simulink model "pioneerSNL"  (R2023b)
settings: Solver=ode23t  StartTime=0  StopTime=1300  FixedStep=0.05  MaxStep=0.05  RelTol=1e-3
values from neighbouring files (symbols this model uses):
  aboveWaterMass = 0    [wecSimInputFile.m]
  L0 = 15+19.8    (= 34.8)    [buildMCR.m]    (also in wecSimInputFile.m)
  polyNom = 1.0e+04*[1.9488   -0.0390   -1.3588    0.8094   -0.0004]    [wecSimInputFile.m]
  simu = simulationClass()    [wecSimInputFile.m]
  waves = waveClass('spectrumImportFullDir')    [wecSimInputFile.m]
undefined symbols (not defined in the file or in its folder): body, cable, constraint, geometry, hydroData, pto, X, Y, Z
libraries: nesl_utility x21, sm_lib x17, WECSim_Lib_Body_Elements x7, WECSim_Lib_PTOs x3, WECSim_Lib_Constraints x2, WECSim_Lib_Cables x1, WECSim_Lib_Moorings x1, WECSim_Lib_Frames x1
(part 1 of 2)
settings Model: Creator=dforbus  LastModifiedBy=jtgrasb
settings SolverCC: ZeroCrossControl=DisableAll  AutoInsertRateTranBlk=on
settings DataIOCC: ReturnWorkspaceOutputs=off
settings OptimizationCC: SimCompilerOptimization=on

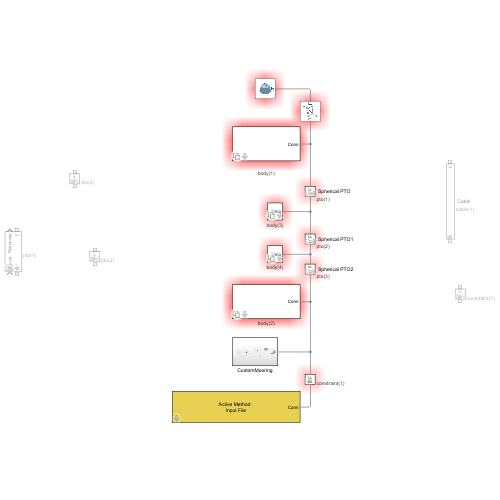
[thumbnail: Simulink's stored preview of the top-level diagram]
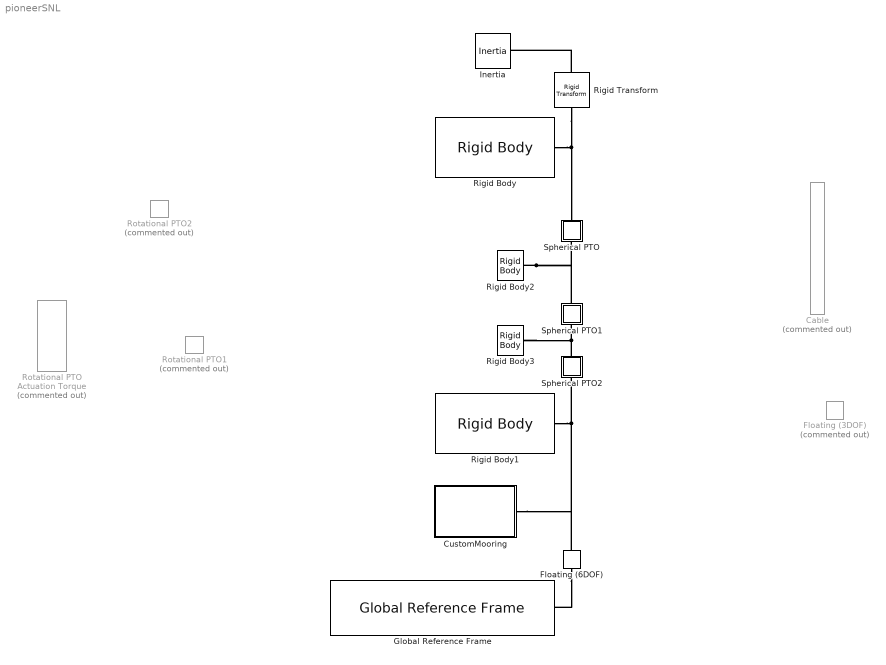
== system pioneerSNL ==
  Cable : WECSim_Lib_Cables/Cable  Commented=on  VariantControl=sv_Cable3DOF  cable=cable(1)  baseConnectionName=constraint(1)  followerConnectionName=constraint(2)  stiffness=0  damping=0  length=0  preTension=0  diplacement=0 0 0  axis=0 1 0  angle=0  y=0 1 0  z=0 0 1
      settings: AttributesFormatString=%<cable>
  CustomMooring : Subsystem
  Floating (3DOF) : WECSim_Lib_Constraints/Floating (3DOF)  Commented=on  constraint=constraint(1)  loc="0  0  0"  displacement=0 0 0  y=0 1 0  z=0 0 1  upperLimitSpecify=off  upperLimitBound=0  upperLimitTransitionRegionWidth=0  upperLimitStiffness=0  upperLimitDamping=0  lowerLimitSpecify=off  lowerLimitBound=0  lowerLimitTransitionRegionWidth=0  lowerLimitStiffness=0  lowerLimitDamping=0
      settings: AttributesFormatString=%<constraint>
  Floating (6DOF) : WECSim_Lib_Constraints/Floating (6DOF)  constraint=constraint(1)  loc="0  0  0"  displacement=0 0 0  y=0 1 0  z=0 0 1  upperLimitSpecify=off  upperLimitBound=0  upperLimitTransitionRegionWidth=0  upperLimitStiffness=0  upperLimitDamping=0  lowerLimitSpecify=off  lowerLimitBound=0  lowerLimitTransitionRegionWidth=0  lowerLimitStiffness=0  lowerLimitDamping=0
      settings: AttributesFormatString=%<constraint>
  Global Reference Frame : WECSim_Lib_Frames/Global Reference Frame  waves=waves  simu=simu  InputMethod=Input File  InputFile=wecSimInputFile.m  mode=normal  explorer=off  solver=ode4  startTime=0  rampTime=100  endTime=400  dt=0.1  cicEndTime=60  stateSpace=0  WaveClass=regular  height=2.5  period=8  elevationFile=NOT DEFINED  spectrumFile=NOT DEFINED  direction=0  spread=1  spectrumType=NOT DEFINED  phaseSeed=0  option=EqualEnergy
  Inertia : sm_lib/Body Elements/Inertia  InertiaType=PointMass  Mass=aboveWaterMass  MassUnits=kg  CenterOfMass=[0 0 0]  CenterOfMassUnits=m  MomentsOfInertia=[1 1 1]  MomentsOfInertiaUnits=kg*m^2  ProductsOfInertia=[0 0 0]  ProductsOfInertiaUnits=kg*m^2  GraphicType=Marker  MarkerShape=Inertia  MarkerSize=20  GraphicVisPropType=SimpleVisualProperties  GraphicDiffuseColor=[0.5 0.5 0.5]  GraphicSpecularColor=[0.5 0.5 0.5 1.0]  GraphicAmbientColor=[0.15 0.15 0.15 1.0]  GraphicEmissiveColor=[0.0 0.0 0.0 1.0]  GraphicShininess=75  GraphicOpacity=1.0
  Rigid Transform : sm_lib/Frames and Transforms/Rigid Transform  TranslationMethod=Cartesian  TranslationStandardOffset=0  TranslationStandardOffsetUnits=m  TranslationStandardAxis=+Z  TranslationCartesianOffset=aboveWaterMassLoc  TranslationCartesianOffsetUnits=m  TranslationROffset=0  TranslationROffsetUnits=m  TranslationZOffset=0  TranslationZOffsetUnits=m  TranslationThetaOffset=0  TranslationThetaOffsetUnits=deg  RotationMethod=None  RotationAngleUnits=deg  RotationStandardAxis=+Z  RotationAngle=0.0  RotationArbitraryAxis=[0 0 1]  FollAlignAxisA=+X  BaseAlignAxisA=+Y  FollAlignAxisB=+Y  BaseAlignAxisB=+Z  RotationSequenceAxes=FollowerAxes  RotationSequence=XYX  RotationSequenceAngles=[0 0 0]  RotationSequenceAnglesUnits=deg  RotationMatrix=[1 0 0; 0 1 0; 0 0 1]  Quaternion=[1 0 0 0]
  Rigid Body : WECSim_Lib_Body_Elements/Rigid Body  body=body(1)  h5File=hydroData/*.h5  geometryFile=geometry/*.stl  mass=0  inertia=0 0 0  inertiaProducts=0 0 0  nonHydro=0  nonlinearHydro=0  centerGravity=0 0 0  centerBuoyancy=0 0 0  dof=6  volume=0  QTFs=0  displacement=0 0 0  axis=0 1 0  angle=0  option=0  cd=0 0 0  ca=0 0 0  area=0 0 0  VME=0  rgME=0 0 0  z=0 0 1
  Rigid Body1 : WECSim_Lib_Body_Elements/Rigid Body  body=body(2)  h5File=hydroData/*.h5  geometryFile=geometry/*.stl  mass=0  inertia=0 0 0  inertiaProducts=0 0 0  nonHydro=0  nonlinearHydro=0  centerGravity=0 0 0  centerBuoyancy=0 0 0  dof=6  volume=0  QTFs=0  displacement=0 0 0  axis=0 1 0  angle=0  option=0  cd=0 0 0  ca=0 0 0  area=0 0 0  VME=0  rgME=0 0 0  z=0 0 1
  Rigid Body2 : WECSim_Lib_Body_Elements/Rigid Body  body=body(3)  h5File=hydroData/*.h5  geometryFile=geometry/*.stl  mass=0  inertia=0 0 0  inertiaProducts=0 0 0  nonHydro=0  nonlinearHydro=0  centerGravity=0 0 0  centerBuoyancy=0 0 0  dof=6  volume=0  QTFs=0  displacement=0 0 0  axis=0 1 0  angle=0  option=0  cd=0 0 0  ca=0 0 0  area=0 0 0  VME=0  rgME=0 0 0  z=0 0 1
  Rigid Body3 : WECSim_Lib_Body_Elements/Rigid Body  body=body(4)  h5File=hydroData/*.h5  geometryFile=geometry/*.stl  mass=0  inertia=0 0 0  inertiaProducts=0 0 0  nonHydro=0  nonlinearHydro=0  centerGravity=0 0 0  centerBuoyancy=0 0 0  dof=6  volume=0  QTFs=0  displacement=0 0 0  axis=0 1 0  angle=0  option=0  cd=0 0 0  ca=0 0 0  area=0 0 0  VME=0  rgME=0 0 0  z=0 0 1
  Rotational PTO Actuation Torque : WECSim_Lib_PTOs/Rotational PTO Actuation Torque  Commented=on  pto=pto(1)  loc="0  0  0"  stiffness=0  damping=0  equilibriumPosition=0  pretension=0  displacement=0 0 0  y=0 1 0  z=0 0 1  upperLimitSpecify=off  upperLimitBound=0  upperLimitTransitionRegionWidth=0  upperLimitStiffness=0  upperLimitDamping=0  lowerLimitSpecify=off  lowerLimitBound=0  lowerLimitTransitionRegionWidth=0  lowerLimitStiffness=0  lowerLimitDamping=0
      settings: AttributesFormatString=%<pto>
  Rotational PTO1 : WECSim_Lib_PTOs/Rotational PTO  Commented=on  pto=pto(2)  loc="0  0  0"  stiffness=0  damping=0  equilibriumPosition=0  pretension=0  displacement=0 0 0  y=0 1 0  z=0 0 1  upperLimitSpecify=off  upperLimitBound=0  upperLimitTransitionRegionWidth=0  upperLimitStiffness=0  upperLimitDamping=0  lowerLimitSpecify=off  lowerLimitBound=0  lowerLimitTransitionRegionWidth=0  lowerLimitStiffness=0  lowerLimitDamping=0
      settings: AttributesFormatString=%<pto>
  Rotational PTO2 : WECSim_Lib_PTOs/Rotational PTO  Commented=on  pto=pto(3)  loc="0  0  0"  stiffness=0  damping=0  equilibriumPosition=0  pretension=0  displacement=0 0 0  y=0 1 0  z=0 0 1  upperLimitSpecify=off  upperLimitBound=0  upperLimitTransitionRegionWidth=0  upperLimitStiffness=0  upperLimitDamping=0  lowerLimitSpecify=off  lowerLimitBound=0  lowerLimitTransitionRegionWidth=0  lowerLimitStiffness=0  lowerLimitDamping=0
      settings: AttributesFormatString=%<pto>
  Spherical PTO : Subsystem  AncestorBlock=WECSim_Lib_PTOs/Spherical PTO  mask(PTOs){pto=pto(1), InputFileText=Global Reference Frame option "Use Input File" is selected., loc=[0 0 0], stiffness=0, damping=0, displacement=[0 0 0], x=, y=0 1 0, z=0 0 1, upperLimitSpecify=on, upperLimitBound=0, upperLimitTransitionRegionWidth=0, upperLimitStiffness=0, upperLimitDamping=0, lowerLimitSpecify=on, lowerLimitBound=0, lowerLimitTransitionRegionWidth=0, lowerLimitStiffness=0, lowerLimitDamping=0}
      mask prompts: pto "PTO Name:"; loc "Location [m]:"; stiffness "PTO Stiffness [N/m]"; damping "PTO Damping [N/m/s]"; displacement "Initial linear displacement [m]:"; x "X-axis [m]:"; y "Y-axis [m]:"; z "Z-axis [m]:"; upperLimitSpecify "Upper limit"; upperLimitBound "Upper limit bound [m, deg]"; upperLimitTransitionRegionWidth "Upper limit transition region width [m, deg]:"; upperLimitStiffness "Upper limit stiffness [N/m, Nm/rad]:"; upperLimitDamping "Upper limit damping [N/(m/s), Nm/(rad/s)]:"; lowerLimitSpecify "Lower limit"; lowerLimitBound "Lower limit bound [m, deg]:"; lowerLimitTransitionRegionWidth "Lower limit transition region width [m, deg]:"; lowerLimitStiffness "Lower limit stiffness [N/m, Nm/rad]:"; lowerLimitDamping "Lower limit damping [N/(m/s), Nm/(rad/s)]:"
      mask help:
      | Constrains the follower to rotational motion relative to the base, fixing in
      | X,Y,Z but allowing rotation about each axis and adds PTO stiffness and damping.
      |
      | The variable name input below must be 'pto(i)' where i=1,2,...
      | pto(i) must be defined in the input file with the following fields:
      |
      |     .name (required)
      |             String.
      |            Constraint name. Must comply with Matlab's variable naming rules.
      |     .location (optional)
      |             3x1 vector [x y z] in meters.
      |             Constraint location. Default = [0 0 0]
      |     .stiffness (optional)
      |             Float.
      |             PTO linear spring stiffness. Default = 0
      |     .damping (optional)
      |             Float.
      |             PTO linear damping coefficient. Default = 0
      |     .orientation.z (optional)
      |             3x1 vector [x y z].
      |             Direction of the constraint's Z-coordinate. Default = [0 0 1]
      |     .orientation.y (optional)
      |             3x1 vector [x y z].
      |             Direction of the constraint's Y-coordinate. Default = [0 1 0]
      mask init:
      | if exist('pto','var')
      |     h=[gcb '/To Workspace'];
      |     responseName=['pto' num2str(pto.number) '_out'];
      |     set_param(h,'VariableName',responseName);
      |     h=[gcb '/Spherical Joint)'];
      |     try % this should catch any version issue for which these parameters do not exist
      |         set_param(h,'upperLimitSpecify',pto.hardStops.upperLimitSpecify)
      |         set_param(h,'lowerLimitSpecify',pto.hardStops.lowerLimitSpecify)
      |     end
      | end
      | 
      | pto.checkLoc('W');
      settings: AttributesFormatString=%<pto>
      mask Help:
      | Constrains the follower to rotational motion relative to the base, fixing in
      | X,Y,Z but allowing rotation about each axis and adds PTO stiffness and damping.
      | 
      | The variable name input below must be 'pto(i)' where i=1,2,...
      | pto(i) must be defined in the input file with the following fields:
      | 
      |     .name (required)
      |             String.
      |            Constraint name. Must comply with Matlab's variable naming rules.
      |     .location (optional)
      |             3x1 vector [x y z] in meters.
      |             Constraint location. Default = [0 0 0]
      |     .stiffness (optional)
      |             Float.
      |             PTO linear spring stiffness. Default = 0
      |     .damping (optional)
      |             Float.
      |             PTO linear damping coefficient. Default = 0
      |     .orientation.z (optional)
      |             3x1 vector [x y z].
      |             Direction of the constraint's Z-coordinate. Default = [0 0 1]
      |     .orientation.y (optional)
      |             3x1 vector [x y z].
      |             Direction of the constraint's Y-coordinate. Default = [0 1 0]
      mask Callback upperLimitSpecify: hardStopCallback(gcbh)
      mask Callback lowerLimitSpecify: hardStopCallback(gcbh)
      mask DialogControl InputFileGroup Prompt: Input File
      mask DialogControl CustomParameterGroup Prompt: Custom Parameters
      mask DialogControl std_opts Prompt: Standard options
      mask DialogControl orientations Prompt: Orientation
      mask DialogControl Container7 Prompt: Hard stop
  Spherical PTO1 : Subsystem  AncestorBlock=WECSim_Lib_PTOs/Spherical PTO  mask(PTOs){pto=pto(2), InputFileText=Global Reference Frame option "Use Input File" is selected., loc=[0 0 0], stiffness=0, damping=0, displacement=[0 0 0], x=, y=0 1 0, z=0 0 1, upperLimitSpecify=on, upperLimitBound=0, upperLimitTransitionRegionWidth=0, upperLimitStiffness=0, upperLimitDamping=0, lowerLimitSpecify=on, lowerLimitBound=0, lowerLimitTransitionRegionWidth=0, lowerLimitStiffness=0, lowerLimitDamping=0}
      mask prompts: pto "PTO Name:"; loc "Location [m]:"; stiffness "PTO Stiffness [N/m]"; damping "PTO Damping [N/m/s]"; displacement "Initial linear displacement [m]:"; x "X-axis [m]:"; y "Y-axis [m]:"; z "Z-axis [m]:"; upperLimitSpecify "Upper limit"; upperLimitBound "Upper limit bound [m, deg]"; upperLimitTransitionRegionWidth "Upper limit transition region width [m, deg]:"; upperLimitStiffness "Upper limit stiffness [N/m, Nm/rad]:"; upperLimitDamping "Upper limit damping [N/(m/s), Nm/(rad/s)]:"; lowerLimitSpecify "Lower limit"; lowerLimitBound "Lower limit bound [m, deg]:"; lowerLimitTransitionRegionWidth "Lower limit transition region width [m, deg]:"; lowerLimitStiffness "Lower limit stiffness [N/m, Nm/rad]:"; lowerLimitDamping "Lower limit damping [N/(m/s), Nm/(rad/s)]:"
      mask help:
      | Constrains the follower to rotational motion relative to the base, fixing in
      | X,Y,Z but allowing rotation about each axis and adds PTO stiffness and damping.
      |
      | The variable name input below must be 'pto(i)' where i=1,2,...
      | pto(i) must be defined in the input file with the following fields:
      |
      |     .name (required)
      |             String.
      |            Constraint name. Must comply with Matlab's variable naming rules.
      |     .location (optional)
      |             3x1 vector [x y z] in meters.
      |             Constraint location. Default = [0 0 0]
      |     .stiffness (optional)
      |             Float.
      |             PTO linear spring stiffness. Default = 0
      |     .damping (optional)
      |             Float.
      |             PTO linear damping coefficient. Default = 0
      |     .orientation.z (optional)
      |             3x1 vector [x y z].
      |             Direction of the constraint's Z-coordinate. Default = [0 0 1]
      |     .orientation.y (optional)
      |             3x1 vector [x y z].
      |             Direction of the constraint's Y-coordinate. Default = [0 1 0]
      mask init: same as pioneerSNL/Spherical PTO
      settings: AttributesFormatString=%<pto>
      mask Help:
      | Constrains the follower to rotational motion relative to the base, fixing in
      | X,Y,Z but allowing rotation about each axis and adds PTO stiffness and damping.
      | 
      | The variable name input below must be 'pto(i)' where i=1,2,...
      | pto(i) must be defined in the input file with the following fields:
      | 
      |     .name (required)
      |             String.
      |            Constraint name. Must comply with Matlab's variable naming rules.
      |     .location (optional)
      |             3x1 vector [x y z] in meters.
      |             Constraint location. Default = [0 0 0]
      |     .stiffness (optional)
      |             Float.
      |             PTO linear spring stiffness. Default = 0
      |     .damping (optional)
      |             Float.
      |             PTO linear damping coefficient. Default = 0
      |     .orientation.z (optional)
      |             3x1 vector [x y z].
      |             Direction of the constraint's Z-coordinate. Default = [0 0 1]
      |     .orientation.y (optional)
      |             3x1 vector [x y z].
      |             Direction of the constraint's Y-coordinate. Default = [0 1 0]
      mask Callback upperLimitSpecify: hardStopCallback(gcbh)
      mask Callback lowerLimitSpecify: hardStopCallback(gcbh)
      mask DialogControl InputFileGroup Prompt: Input File
      mask DialogControl CustomParameterGroup Prompt: Custom Parameters
      mask DialogControl std_opts Prompt: Standard options
      mask DialogControl orientations Prompt: Orientation
      mask DialogControl Container7 Prompt: Hard stop
  Spherical PTO2 : Subsystem  AncestorBlock=WECSim_Lib_PTOs/Spherical PTO  mask(PTOs){pto=pto(3), InputFileText=Global Reference Frame option "Use Input File" is selected., loc=[0 0 0], stiffness=0, damping=0, displacement=[0 0 0], x=, y=0 1 0, z=0 0 1, upperLimitSpecify=on, upperLimitBound=0, upperLimitTransitionRegionWidth=0, upperLimitStiffness=0, upperLimitDamping=0, lowerLimitSpecify=on, lowerLimitBound=0, lowerLimitTransitionRegionWidth=0, lowerLimitStiffness=0, lowerLimitDamping=0}
      mask prompts: pto "PTO Name:"; loc "Location [m]:"; stiffness "PTO Stiffness [N/m]"; damping "PTO Damping [N/m/s]"; displacement "Initial linear displacement [m]:"; x "X-axis [m]:"; y "Y-axis [m]:"; z "Z-axis [m]:"; upperLimitSpecify "Upper limit"; upperLimitBound "Upper limit bound [m, deg]"; upperLimitTransitionRegionWidth "Upper limit transition region width [m, deg]:"; upperLimitStiffness "Upper limit stiffness [N/m, Nm/rad]:"; upperLimitDamping "Upper limit damping [N/(m/s), Nm/(rad/s)]:"; lowerLimitSpecify "Lower limit"; lowerLimitBound "Lower limit bound [m, deg]:"; lowerLimitTransitionRegionWidth "Lower limit transition region width [m, deg]:"; lowerLimitStiffness "Lower limit stiffness [N/m, Nm/rad]:"; lowerLimitDamping "Lower limit damping [N/(m/s), Nm/(rad/s)]:"
      mask help:
      | Constrains the follower to rotational motion relative to the base, fixing in
      | X,Y,Z but allowing rotation about each axis and adds PTO stiffness and damping.
      |
      | The variable name input below must be 'pto(i)' where i=1,2,...
      | pto(i) must be defined in the input file with the following fields:
      |
      |     .name (required)
      |             String.
      |            Constraint name. Must comply with Matlab's variable naming rules.
      |     .location (optional)
      |             3x1 vector [x y z] in meters.
      |             Constraint location. Default = [0 0 0]
      |     .stiffness (optional)
      |             Float.
      |             PTO linear spring stiffness. Default = 0
      |     .damping (optional)
      |             Float.
      |             PTO linear damping coefficient. Default = 0
      |     .orientation.z (optional)
      |             3x1 vector [x y z].
      |             Direction of the constraint's Z-coordinate. Default = [0 0 1]
      |     .orientation.y (optional)
      |             3x1 vector [x y z].
      |             Direction of the constraint's Y-coordinate. Default = [0 1 0]
      mask init: same as pioneerSNL/Spherical PTO
      settings: AttributesFormatString=%<pto>
      mask Help:
      | Constrains the follower to rotational motion relative to the base, fixing in
      | X,Y,Z but allowing rotation about each axis and adds PTO stiffness and damping.
      | 
      | The variable name input below must be 'pto(i)' where i=1,2,...
      | pto(i) must be defined in the input file with the following fields:
      | 
      |     .name (required)
      |             String.
      |            Constraint name. Must comply with Matlab's variable naming rules.
      |     .location (optional)
      |             3x1 vector [x y z] in meters.
      |             Constraint location. Default = [0 0 0]
      |     .stiffness (optional)
      |             Float.
      |             PTO linear spring stiffness. Default = 0
      |     .damping (optional)
      |             Float.
      |             PTO linear damping coefficient. Default = 0
      |     .orientation.z (optional)
      |             3x1 vector [x y z].
      |             Direction of the constraint's Z-coordinate. Default = [0 0 1]
      |     .orientation.y (optional)
      |             3x1 vector [x y z].
      |             Direction of the constraint's Y-coordinate. Default = [0 1 0]
      mask Callback upperLimitSpecify: hardStopCallback(gcbh)
      mask Callback lowerLimitSpecify: hardStopCallback(gcbh)
      mask DialogControl InputFileGroup Prompt: Input File
      mask DialogControl CustomParameterGroup Prompt: Custom Parameters
      mask DialogControl std_opts Prompt: Standard options
      mask DialogControl orientations Prompt: Orientation
      mask DialogControl Container7 Prompt: Hard stop
  connections:
  Rigid Body2/RConn1 -- Spherical PTO1/RConn1 -- Spherical PTO/LConn1
  Rigid Body/RConn1 -- Spherical PTO/RConn1 -- Rigid Transform/LConn1
  Rigid Body3/RConn1 -- Spherical PTO2/RConn1 -- Spherical PTO1/LConn1
  Rigid Body1/RConn1 -- CustomMooring/LConn1 -- Floating (6DOF)/RConn1 -- Spherical PTO2/LConn1
  Floating (6DOF)/LConn1 -- Global Reference Frame/RConn1
  Rigid Transform/RConn1 -- Inertia/RConn1

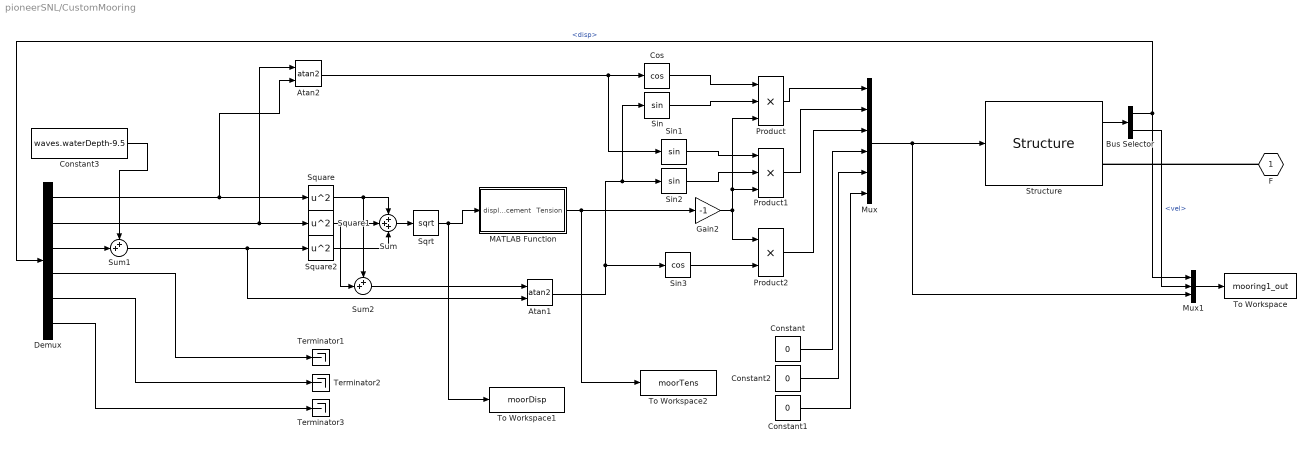
== system pioneerSNL/CustomMooring ==
  Atan1 : Trigonometry  Operator=atan2
  Atan2 : Trigonometry  Operator=atan2
  Bus Selector : BusSelector  OutputSignals=disp,vel
  Constant : Constant  Value=0
  Constant1 : Constant  Value=0
  Constant2 : Constant  Value=0
  Constant3 : Constant  Value=waves.waterDepth-9.5
  Cos : Trigonometry  Operator=cos
  Demux : Demux  Outputs=6
  Gain2 : Gain  Gain=-1
  MATLAB Function : MATLAB Function  TreatAsAtomicUnit=on
  Mux : Mux  Inputs=6
  Mux1 : Mux  Inputs=3
  Product : Product  Inputs=3
  Product1 : Product  Inputs=3
  Product2 : Product
  Sin : Trigonometry
  Sin1 : Trigonometry
  Sin2 : Trigonometry
  Sin3 : Trigonometry  Operator=cos
  Sqrt : Sqrt
  Square : Math  Operator=square
  Square1 : Math  Operator=square
  Square2 : Math  Operator=square
  Structure : WECSim_Lib_Moorings/MooringMatrix/Structure  SystemSampleTime=-1  VariantActivationTime=update diagram  AllowFlexibleInterface=on  Latency=0  AutoFrameSizeCalculation=off
      link override Body Properties: SerializedExposedGeometries=<exposedGeometries/>
  Sum : Sum  Inputs=+++
  Sum1 : Sum  Inputs=++|
  Sum2 : Sum  Inputs=++|
  Terminator1 : Terminator
  Terminator2 : Terminator
  Terminator3 : Terminator
  To Workspace : ToWorkspace  VariableName=mooring1_out  SaveFormat=Structure With Time  SampleTime=simu.dtOut
  To Workspace1 : ToWorkspace  VariableName=moorDisp  SaveFormat=Timeseries  SampleTime=-1
  To Workspace2 : ToWorkspace  VariableName=moorTens  SaveFormat=Timeseries  SampleTime=-1
  F : PMIOPort  Side=Left
  wires:
  Sqrt/1 -> To Workspace1/1, MATLAB Function/1(displacement)
  Demux/6 -> Terminator3/1
  Constant/1 -> Mux/4
  Sin/1 -> Product/2
  Sin2/1 -> Product1/2
  Constant2/1 -> Mux/5
  Product1/1 -> Mux/2
  Product/1 -> Mux/1
  Demux/4 -> Terminator1/1
  Demux/5 -> Terminator2/1
  Constant1/1 -> Mux/6
  Cos/1 -> Product/1
  Sin1/1 -> Product1/1
  Sum/1 -> Sqrt/1
  Mux1/1 -> To Workspace/1
  Structure/1 -> Bus Selector/1
  Bus Selector/1 -> Demux/1, Mux1/1  "<disp>"
  Bus Selector/2 -> Mux1/2  "<vel>"
  Atan2/1 -> Sin1/1, Cos/1
  Atan1/1 -> Sin3/1, Sin2/1, Sin/1
  Product2/1 -> Mux/3
  Square2/1 -> Sum/3
  Square1/1 -> Sum/2, Sum2/2
  Square/1 -> Sum2/1, Sum/1
  Sum1/1 -> Square2/1, Atan1/2
  Demux/3 -> Sum1/2
  Constant3/1 -> Sum1/1
  Demux/2 -> Square1/1, Atan2/1
  MATLAB Function/1(Tension) -> To Workspace2/1, Gain2/1
  Sum2/1 -> Atan1/1
  Mux/1 -> Structure/1, Mux1/3
  Demux/1 -> Square/1, Atan2/2
  Gain2/1 -> Product/3, Product1/3, Product2/1
  Sin3/1 -> Product2/2
  connections:
  F/RConn1 -- Structure/RConn1

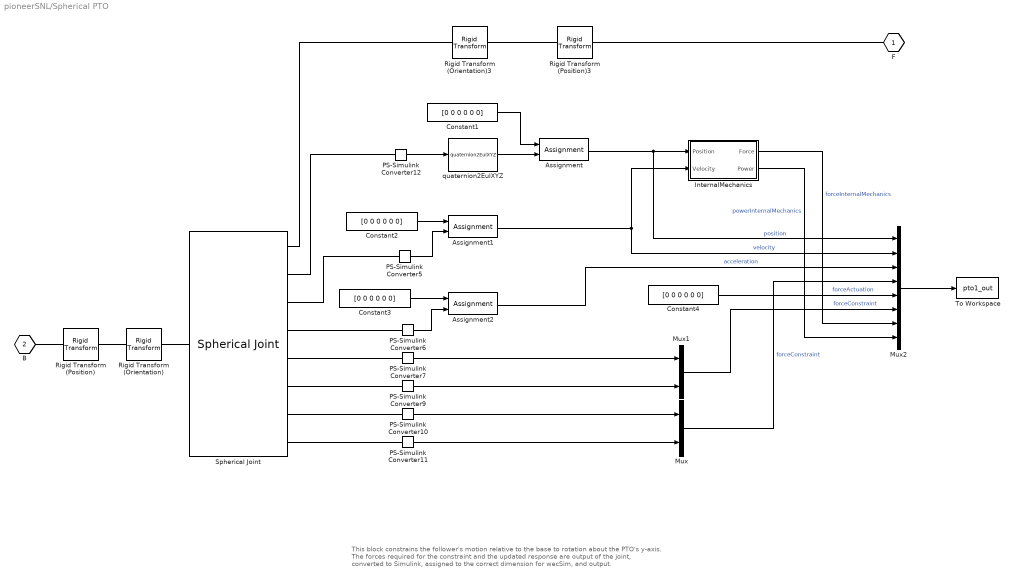
== system pioneerSNL/Spherical PTO ==
  note: This block constrains the follower's motion relative to the base to rotation about the PTO's y-axis. The forces required for the constraint and the updated response are output of the joint, converted to Simulink, assigned to the correct dimension for wecSim, and output.
  Assignment : Assignment  IndexOptions=Index vector (dialog)  Indices=[4 5 6]  OutputSizes=1
  Assignment1 : Assignment  IndexOptions=Index vector (dialog)  Indices=[4 5 6]  OutputSizes=1
  Assignment2 : Assignment  IndexOptions=Index vector (dialog)  Indices=[4,5,6]  OutputSizes=1
  Constant{1..4} (4 alike) : Constant  Value=[0 0 0 0 0 0]
  InternalMechanics : Subsystem
  Mux : Mux  Inputs=2
  Mux1 : Mux  Inputs=2
  Mux2 : Mux  Inputs=8
  PS-Simulink Converter{5..7,9..12} (7 alike) : nesl_utility/PS-Simulink Converter  PhysicalDomain=network_engine_domain  SubClassName=ps_output  LeftPortType=input  RightPortType=output  PseudoPeriodic=off  Frequencies=[]  VectorFormat=1-D array  Unit=inherit  AffineConversion=off
  Rigid Transform (Orientation) : sm_lib/Frames and Transforms/Rigid Transform  TranslationMethod=None  TranslationStandardOffset=0  TranslationStandardOffsetUnits=m  TranslationStandardAxis=+Z  TranslationCartesianOffset=constraint.initial.displacement+constraint.location  TranslationCartesianOffsetUnits=m  TranslationROffset=0  TranslationROffsetUnits=m  TranslationZOffset=0  TranslationZOffsetUnits=m  TranslationThetaOffset=0  TranslationThetaOffsetUnits=deg  RotationMethod=RotationMatrix  RotationAngleUnits=deg  RotationStandardAxis=+Z  RotationAngle=0.0  RotationArbitraryAxis=[0 0 1]  FollAlignAxisA=+X  BaseAlignAxisA=+Y  FollAlignAxisB=+Y  BaseAlignAxisB=+Z  RotationSequenceAxes=FollowerAxes  RotationSequence=XYX  RotationSequenceAngles=[0 0 0]  RotationSequenceAnglesUnits=deg  RotationMatrix=pto.orientation.rotationMatrix  Quaternion=[1 0 0 0]
  Rigid Transform (Orientation)3 : sm_lib/Frames and Transforms/Rigid Transform  TranslationMethod=None  TranslationStandardOffset=0  TranslationStandardOffsetUnits=m  TranslationStandardAxis=+Z  TranslationCartesianOffset=constraint.initial.displacement+constraint.location  TranslationCartesianOffsetUnits=m  TranslationROffset=0  TranslationROffsetUnits=m  TranslationZOffset=0  TranslationZOffsetUnits=m  TranslationThetaOffset=0  TranslationThetaOffsetUnits=deg  RotationMethod=RotationMatrix  RotationAngleUnits=deg  RotationStandardAxis=+Z  RotationAngle=0.0  RotationArbitraryAxis=[0 0 1]  FollAlignAxisA=+X  BaseAlignAxisA=+Y  FollAlignAxisB=+Y  BaseAlignAxisB=+Z  RotationSequenceAxes=FollowerAxes  RotationSequence=XYX  RotationSequenceAngles=[0 0 0]  RotationSequenceAnglesUnits=deg  RotationMatrix=pto.orientation.rotationMatrix  Quaternion=[1 0 0 0]
  Rigid Transform (Position) : sm_lib/Frames and Transforms/Rigid Transform  TranslationMethod=Cartesian  TranslationStandardOffset=0  TranslationStandardOffsetUnits=m  TranslationStandardAxis=+Z  TranslationCartesianOffset=pto.initial.displacement+pto.location  TranslationCartesianOffsetUnits=m  TranslationROffset=0  TranslationROffsetUnits=m  TranslationZOffset=0  TranslationZOffsetUnits=m  TranslationThetaOffset=0  TranslationThetaOffsetUnits=deg  RotationMethod=None  RotationAngleUnits=deg  RotationStandardAxis=+Z  RotationAngle=0.0  RotationArbitraryAxis=[0 0 1]  FollAlignAxisA=+X  BaseAlignAxisA=+Y  FollAlignAxisB=+Y  BaseAlignAxisB=+Z  RotationSequenceAxes=FollowerAxes  RotationSequence=XYX  RotationSequenceAngles=[0 0 0]  RotationSequenceAnglesUnits=deg  RotationMatrix=[1 0 0; 0 1 0; 0 0 1]  Quaternion=[1 0 0 0]
  Rigid Transform (Position)3 : sm_lib/Frames and Transforms/Rigid Transform  TranslationMethod=Cartesian  TranslationStandardOffset=0  TranslationStandardOffsetUnits=m  TranslationStandardAxis=+Z  TranslationCartesianOffset=pto.initial.displacement+pto.location  TranslationCartesianOffsetUnits=m  TranslationROffset=0  TranslationROffsetUnits=m  TranslationZOffset=0  TranslationZOffsetUnits=m  TranslationThetaOffset=0  TranslationThetaOffsetUnits=deg  RotationMethod=None  RotationAngleUnits=deg  RotationStandardAxis=+Z  RotationAngle=0.0  RotationArbitraryAxis=[0 0 1]  FollAlignAxisA=+X  BaseAlignAxisA=+Y  FollAlignAxisB=+Y  BaseAlignAxisB=+Z  RotationSequenceAxes=FollowerAxes  RotationSequence=XYX  RotationSequenceAngles=[0 0 0]  RotationSequenceAnglesUnits=deg  RotationMatrix=[1 0 0; 0 1 0; 0 0 1]  Quaternion=[1 0 0 0]
  Spherical Joint : sm_lib/Joints/Spherical Joint  JointMode=Normal  SenseConstraintForce=on  SenseConstraintForceX=off  SenseConstraintForceY=off  SenseConstraintForceZ=off  SenseConstraintTorque=on  SenseConstraintTorqueX=off  SenseConstraintTorqueY=off  SenseConstraintTorqueZ=off  SenseTotalForce=on  SenseTotalForceX=off  SenseTotalForceY=off  SenseTotalForceZ=off  SenseTotalTorque=on  SenseTotalTorqueX=off  SenseTotalTorqueY=off  SenseTotalTorqueZ=off  CompositeWrenchDir=BaseOnFollower  CompositeWrenchFrame=BaseFrame  EqPosRotationMethod=None  EqPosRotationAngleUnits=deg  EqPosRotationStandardAxis=+Z  EqPosRotationAngle=0.0  EqPosRotationArbitraryAxis=[0 0 1]  EqPosFollAlignAxisA=+X  EqPosBaseAlignAxisA=+Y  EqPosFollAlignAxisB=+Y  EqPosBaseAlignAxisB=+Z  EqPosRotationSequenceAxes=FollowerAxes  EqPosRotationSequence=XYX  EqPosRotationSequenceAngles=[0 0 0]  EqPosRotationSequenceAnglesUnits=deg  EqPosRotationMatrix=[1 0 0; 0 1 0; 0 0 1]  EqPosQuaternion=[1 0 0 0]  SpringStiffness=pto.stiffness  SpringStiffnessUnits=N*m/rad  DampingCoefficient=pto.damping  DampingCoefficientUnits=N*m/(rad/s)  ActuateTorqueX=off  ActuateTorqueY=off  ActuateTorqueZ=off  ActuateTorque=off  TorqueActuationMode=NoTorque  MotionActuationMode=ComputedMotion  ActuationFrame=BaseFrame  SensePosition=on  SenseVelocityX=off  SenseVelocityY=off  SenseVelocityZ=off  SenseVelocity=on  SenseAccelerationX=off  SenseAccelerationY=off  SenseAccelerationZ=off  SenseAcceleration=on  SenseTorqueX=off  SenseTorqueY=off  SenseTorqueZ=off  SenseTorqueForce=off  SenseLowerLimitTorqueMag=off  SenseUpperLimitTorqueMag=off  SensingFrame=BaseFrame  LowerLimitSpecify=off  LowerLimitBound=15  LowerLimitBoundUnits=deg  LowerLimitStiffness=1e4  LowerLimitStiffnessUnits=N*m/deg  LowerLimitDamping=10  LowerLimitDampingUnits=N*m/(deg/s)  LowerLimitTransitionRegionWidth=0.1  LowerLimitTransitionRegionWidthUnits=deg  UpperLimitSpecify=off  UpperLimitBound=45  UpperLimitBoundUnits=deg  UpperLimitStiffness=1e4  UpperLimitStiffnessUnits=N*m/deg  UpperLimitDamping=10  UpperLimitDampingUnits=N*m/(deg/s)  UpperLimitTransitionRegionWidth=0.1  UpperLimitTransitionRegionWidthUnits=deg  PositionTargetRotationMethod=None  PositionTargetRotationAngleUnits=deg  PositionTargetRotationStandardAxis=+Z  PositionTargetRotationAngle=0.0  PositionTargetRotationArbitraryAxis=[0 0 1]  PositionTargetFollAlignAxisA=+X  PositionTargetBaseAlignAxisA=+Y  PositionTargetFollAlignAxisB=+Y  PositionTargetBaseAlignAxisB=+Z  PositionTargetRotationSequenceAxes=FollowerAxes  PositionTargetRotationSequence=XYX  PositionTargetRotationSequenceAngles=[0 0 0]  PositionTargetRotationSequenceAnglesUnits=deg  PositionTargetRotationMatrix=[1 0 0; 0 1 0; 0 0 1]  PositionTargetQuaternion=[1 0 0 0]  PositionTargetSpecify=off  PositionTargetPriority=High  VelocityTargetValue=[0 0 0]  VelocityTargetValueUnits=deg/s  VelocityTargetSpecify=off  VelocityTargetPriority=High  VelocityTargetInFollowerFrame=on
  To Workspace : ToWorkspace  VariableName=pto1_out  SaveFormat=Structure With Time  SampleTime=simu.dtOut
  quaternion2EulXYZ : WECSim_Lib_Body_Elements/Rigid Body/Hydrodynamic Body/Structure/Motion Sensor/quaternion2EulXYZ  SystemSampleTime=-1  VariantActivationTime=update diagram  AllowFlexibleInterface=on  Latency=0  AutoFrameSizeCalculation=off
  F : PMIOPort  Side=Right
  B : PMIOPort  Port=2  Side=Left
  wires:
  Mux/1 -> Mux2/4  "forceConstraint"
  Assignment2/1 -> Mux2/3  "acceleration"
  PS-Simulink Converter11/1 -> Mux/2
  PS-Simulink Converter12/1 -> quaternion2EulXYZ/1
  Constant3/1 -> Assignment2/1
  InternalMechanics/2(Power) -> Mux2/8  "powerInternalMechanics"
  Assignment1/1 -> Mux2/2, InternalMechanics/2(Velocity)  "velocity"
  Constant2/1 -> Assignment1/1
  Constant4/1 -> Mux2/5  "forceActuation"
  PS-Simulink Converter6/1 -> Assignment2/2
  Assignment/1 -> Mux2/1, InternalMechanics/1(Position)  "position"
  PS-Simulink Converter7/1 -> Mux1/1
  PS-Simulink Converter10/1 -> Mux/1
  PS-Simulink Converter5/1 -> Assignment1/2
  PS-Simulink Converter9/1 -> Mux1/2
  quaternion2EulXYZ/1 -> Assignment/2
  Constant1/1 -> Assignment/1
  Mux2/1 -> To Workspace/1
  InternalMechanics/1(Force) -> Mux2/7  "forceInternalMechanics"
  Mux1/1 -> Mux2/6  "forceConstraint"
  connections:
  Rigid Transform (Orientation)/RConn1 -- Spherical Joint/LConn1
  Spherical Joint/RConn8 -- PS-Simulink Converter11/LConn1
  Spherical Joint/RConn2 -- PS-Simulink Converter12/LConn1
  Spherical Joint/RConn7 -- PS-Simulink Converter10/LConn1
  Rigid Transform (Orientation)3/LConn1 -- Rigid Transform (Position)3/RConn1
  Rigid Transform (Position)/LConn1 -- B/RConn1
  Spherical Joint/RConn4 -- PS-Simulink Converter6/LConn1
  Spherical Joint/RConn5 -- PS-Simulink Converter7/LConn1
  Spherical Joint/RConn1 -- Rigid Transform (Orientation)3/RConn1
  Rigid Transform (Orientation)/LConn1 -- Rigid Transform (Position)/RConn1
  Spherical Joint/RConn6 -- PS-Simulink Converter9/LConn1
  Rigid Transform (Position)3/LConn1 -- F/RConn1
  Spherical Joint/RConn3 -- PS-Simulink Converter5/LConn1

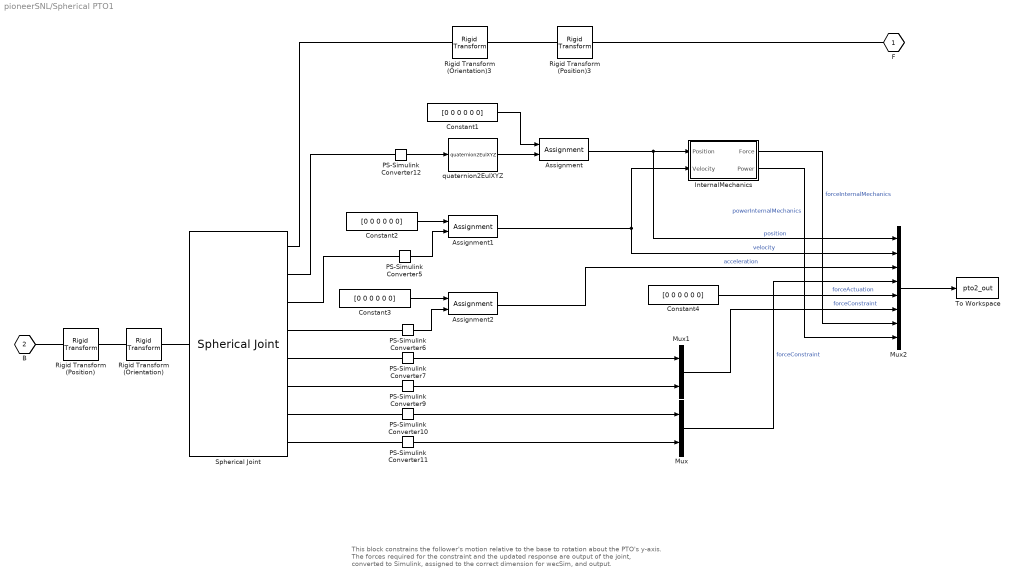
== system pioneerSNL/Spherical PTO1 ==
  note: This block constrains the follower's motion relative to the base to rotation about the PTO's y-axis. The forces required for the constraint and the updated response are output of the joint, converted to Simulink, assigned to the correct dimension for wecSim, and output.
  Assignment : Assignment  IndexOptions=Index vector (dialog)  Indices=[4 5 6]  OutputSizes=1
  Assignment1 : Assignment  IndexOptions=Index vector (dialog)  Indices=[4 5 6]  OutputSizes=1
  Assignment2 : Assignment  IndexOptions=Index vector (dialog)  Indices=[4,5,6]  OutputSizes=1
  Constant{1..4} (4 alike) : Constant  Value=[0 0 0 0 0 0]
  InternalMechanics : Subsystem
  Mux : Mux  Inputs=2
  Mux1 : Mux  Inputs=2
  Mux2 : Mux  Inputs=8
  PS-Simulink Converter{5..7,9..12} (7 alike) : nesl_utility/PS-Simulink Converter  PhysicalDomain=network_engine_domain  SubClassName=ps_output  LeftPortType=input  RightPortType=output  PseudoPeriodic=off  Frequencies=[]  VectorFormat=1-D array  Unit=inherit  AffineConversion=off
  Rigid Transform (Orientation) : sm_lib/Frames and Transforms/Rigid Transform  TranslationMethod=None  TranslationStandardOffset=0  TranslationStandardOffsetUnits=m  TranslationStandardAxis=+Z  TranslationCartesianOffset=constraint.initial.displacement+constraint.location  TranslationCartesianOffsetUnits=m  TranslationROffset=0  TranslationROffsetUnits=m  TranslationZOffset=0  TranslationZOffsetUnits=m  TranslationThetaOffset=0  TranslationThetaOffsetUnits=deg  RotationMethod=RotationMatrix  RotationAngleUnits=deg  RotationStandardAxis=+Z  RotationAngle=0.0  RotationArbitraryAxis=[0 0 1]  FollAlignAxisA=+X  BaseAlignAxisA=+Y  FollAlignAxisB=+Y  BaseAlignAxisB=+Z  RotationSequenceAxes=FollowerAxes  RotationSequence=XYX  RotationSequenceAngles=[0 0 0]  RotationSequenceAnglesUnits=deg  RotationMatrix=pto.orientation.rotationMatrix  Quaternion=[1 0 0 0]
  Rigid Transform (Orientation)3 : sm_lib/Frames and Transforms/Rigid Transform  TranslationMethod=None  TranslationStandardOffset=0  TranslationStandardOffsetUnits=m  TranslationStandardAxis=+Z  TranslationCartesianOffset=constraint.initial.displacement+constraint.location  TranslationCartesianOffsetUnits=m  TranslationROffset=0  TranslationROffsetUnits=m  TranslationZOffset=0  TranslationZOffsetUnits=m  TranslationThetaOffset=0  TranslationThetaOffsetUnits=deg  RotationMethod=RotationMatrix  RotationAngleUnits=deg  RotationStandardAxis=+Z  RotationAngle=0.0  RotationArbitraryAxis=[0 0 1]  FollAlignAxisA=+X  BaseAlignAxisA=+Y  FollAlignAxisB=+Y  BaseAlignAxisB=+Z  RotationSequenceAxes=FollowerAxes  RotationSequence=XYX  RotationSequenceAngles=[0 0 0]  RotationSequenceAnglesUnits=deg  RotationMatrix=pto.orientation.rotationMatrix  Quaternion=[1 0 0 0]
  Rigid Transform (Position) : sm_lib/Frames and Transforms/Rigid Transform  TranslationMethod=Cartesian  TranslationStandardOffset=0  TranslationStandardOffsetUnits=m  TranslationStandardAxis=+Z  TranslationCartesianOffset=pto.initial.displacement+pto.location  TranslationCartesianOffsetUnits=m  TranslationROffset=0  TranslationROffsetUnits=m  TranslationZOffset=0  TranslationZOffsetUnits=m  TranslationThetaOffset=0  TranslationThetaOffsetUnits=deg  RotationMethod=None  RotationAngleUnits=deg  RotationStandardAxis=+Z  RotationAngle=0.0  RotationArbitraryAxis=[0 0 1]  FollAlignAxisA=+X  BaseAlignAxisA=+Y  FollAlignAxisB=+Y  BaseAlignAxisB=+Z  RotationSequenceAxes=FollowerAxes  RotationSequence=XYX  RotationSequenceAngles=[0 0 0]  RotationSequenceAnglesUnits=deg  RotationMatrix=[1 0 0; 0 1 0; 0 0 1]  Quaternion=[1 0 0 0]
  Rigid Transform (Position)3 : sm_lib/Frames and Transforms/Rigid Transform  TranslationMethod=Cartesian  TranslationStandardOffset=0  TranslationStandardOffsetUnits=m  TranslationStandardAxis=+Z  TranslationCartesianOffset=pto.initial.displacement+pto.location  TranslationCartesianOffsetUnits=m  TranslationROffset=0  TranslationROffsetUnits=m  TranslationZOffset=0  TranslationZOffsetUnits=m  TranslationThetaOffset=0  TranslationThetaOffsetUnits=deg  RotationMethod=None  RotationAngleUnits=deg  RotationStandardAxis=+Z  RotationAngle=0.0  RotationArbitraryAxis=[0 0 1]  FollAlignAxisA=+X  BaseAlignAxisA=+Y  FollAlignAxisB=+Y  BaseAlignAxisB=+Z  RotationSequenceAxes=FollowerAxes  RotationSequence=XYX  RotationSequenceAngles=[0 0 0]  RotationSequenceAnglesUnits=deg  RotationMatrix=[1 0 0; 0 1 0; 0 0 1]  Quaternion=[1 0 0 0]
  Spherical Joint : sm_lib/Joints/Spherical Joint  JointMode=Normal  SenseConstraintForce=on  SenseConstraintForceX=off  SenseConstraintForceY=off  SenseConstraintForceZ=off  SenseConstraintTorque=on  SenseConstraintTorqueX=off  SenseConstraintTorqueY=off  SenseConstraintTorqueZ=off  SenseTotalForce=on  SenseTotalForceX=off  SenseTotalForceY=off  SenseTotalForceZ=off  SenseTotalTorque=on  SenseTotalTorqueX=off  SenseTotalTorqueY=off  SenseTotalTorqueZ=off  CompositeWrenchDir=BaseOnFollower  CompositeWrenchFrame=BaseFrame  EqPosRotationMethod=None  EqPosRotationAngleUnits=deg  EqPosRotationStandardAxis=+Z  EqPosRotationAngle=0.0  EqPosRotationArbitraryAxis=[0 0 1]  EqPosFollAlignAxisA=+X  EqPosBaseAlignAxisA=+Y  EqPosFollAlignAxisB=+Y  EqPosBaseAlignAxisB=+Z  EqPosRotationSequenceAxes=FollowerAxes  EqPosRotationSequence=XYX  EqPosRotationSequenceAngles=[0 0 0]  EqPosRotationSequenceAnglesUnits=deg  EqPosRotationMatrix=[1 0 0; 0 1 0; 0 0 1]  EqPosQuaternion=[1 0 0 0]  SpringStiffness=pto.stiffness  SpringStiffnessUnits=N*m/rad  DampingCoefficient=pto.damping  DampingCoefficientUnits=N*m/(rad/s)  ActuateTorqueX=off  ActuateTorqueY=off  ActuateTorqueZ=off  ActuateTorque=off  TorqueActuationMode=NoTorque  MotionActuationMode=ComputedMotion  ActuationFrame=BaseFrame  SensePosition=on  SenseVelocityX=off  SenseVelocityY=off  SenseVelocityZ=off  SenseVelocity=on  SenseAccelerationX=off  SenseAccelerationY=off  SenseAccelerationZ=off  SenseAcceleration=on  SenseTorqueX=off  SenseTorqueY=off  SenseTorqueZ=off  SenseTorqueForce=off  SenseLowerLimitTorqueMag=off  SenseUpperLimitTorqueMag=off  SensingFrame=BaseFrame  LowerLimitSpecify=off  LowerLimitBound=15  LowerLimitBoundUnits=deg  LowerLimitStiffness=1e4  LowerLimitStiffnessUnits=N*m/deg  LowerLimitDamping=10  LowerLimitDampingUnits=N*m/(deg/s)  LowerLimitTransitionRegionWidth=0.1  LowerLimitTransitionRegionWidthUnits=deg  UpperLimitSpecify=off  UpperLimitBound=45  UpperLimitBoundUnits=deg  UpperLimitStiffness=1e4  UpperLimitStiffnessUnits=N*m/deg  UpperLimitDamping=10  UpperLimitDampingUnits=N*m/(deg/s)  UpperLimitTransitionRegionWidth=0.1  UpperLimitTransitionRegionWidthUnits=deg  PositionTargetRotationMethod=None  PositionTargetRotationAngleUnits=deg  PositionTargetRotationStandardAxis=+Z  PositionTargetRotationAngle=0.0  PositionTargetRotationArbitraryAxis=[0 0 1]  PositionTargetFollAlignAxisA=+X  PositionTargetBaseAlignAxisA=+Y  PositionTargetFollAlignAxisB=+Y  PositionTargetBaseAlignAxisB=+Z  PositionTargetRotationSequenceAxes=FollowerAxes  PositionTargetRotationSequence=XYX  PositionTargetRotationSequenceAngles=[0 0 0]  PositionTargetRotationSequenceAnglesUnits=deg  PositionTargetRotationMatrix=[1 0 0; 0 1 0; 0 0 1]  PositionTargetQuaternion=[1 0 0 0]  PositionTargetSpecify=off  PositionTargetPriority=High  VelocityTargetValue=[0 0 0]  VelocityTargetValueUnits=deg/s  VelocityTargetSpecify=off  VelocityTargetPriority=High  VelocityTargetInFollowerFrame=on
  To Workspace : ToWorkspace  VariableName=pto2_out  SaveFormat=Structure With Time  SampleTime=simu.dtOut
  quaternion2EulXYZ : WECSim_Lib_Body_Elements/Rigid Body/Hydrodynamic Body/Structure/Motion Sensor/quaternion2EulXYZ  SystemSampleTime=-1  VariantActivationTime=update diagram  AllowFlexibleInterface=on  Latency=0  AutoFrameSizeCalculation=off
  F : PMIOPort  Side=Right
  B : PMIOPort  Port=2  Side=Left
  wires:
  Mux/1 -> Mux2/4  "forceConstraint"
  Assignment2/1 -> Mux2/3  "acceleration"
  PS-Simulink Converter11/1 -> Mux/2
  PS-Simulink Converter12/1 -> quaternion2EulXYZ/1
  Constant3/1 -> Assignment2/1
  InternalMechanics/2(Power) -> Mux2/8  "powerInternalMechanics"
  Assignment1/1 -> Mux2/2, InternalMechanics/2(Velocity)  "velocity"
  Constant2/1 -> Assignment1/1
  Constant4/1 -> Mux2/5  "forceActuation"
  PS-Simulink Converter6/1 -> Assignment2/2
  Assignment/1 -> Mux2/1, InternalMechanics/1(Position)  "position"
  PS-Simulink Converter7/1 -> Mux1/1
  PS-Simulink Converter10/1 -> Mux/1
  PS-Simulink Converter5/1 -> Assignment1/2
  PS-Simulink Converter9/1 -> Mux1/2
  quaternion2EulXYZ/1 -> Assignment/2
  Constant1/1 -> Assignment/1
  Mux2/1 -> To Workspace/1
  InternalMechanics/1(Force) -> Mux2/7  "forceInternalMechanics"
  Mux1/1 -> Mux2/6  "forceConstraint"
  connections:
  Rigid Transform (Orientation)/RConn1 -- Spherical Joint/LConn1
  Spherical Joint/RConn8 -- PS-Simulink Converter11/LConn1
  Spherical Joint/RConn2 -- PS-Simulink Converter12/LConn1
  Spherical Joint/RConn7 -- PS-Simulink Converter10/LConn1
  Rigid Transform (Orientation)3/LConn1 -- Rigid Transform (Position)3/RConn1
  Rigid Transform (Position)/LConn1 -- B/RConn1
  Spherical Joint/RConn4 -- PS-Simulink Converter6/LConn1
  Spherical Joint/RConn5 -- PS-Simulink Converter7/LConn1
  Spherical Joint/RConn1 -- Rigid Transform (Orientation)3/RConn1
  Rigid Transform (Orientation)/LConn1 -- Rigid Transform (Position)/RConn1
  Spherical Joint/RConn6 -- PS-Simulink Converter9/LConn1
  Rigid Transform (Position)3/LConn1 -- F/RConn1
  Spherical Joint/RConn3 -- PS-Simulink Converter5/LConn1
